simulink model "CIFB2"  (R2022b)
settings: Solver=FixedStepDiscrete  StartTime=0.0  StopTime=0.01  RelTol=1e-3
libraries: dspsrcs4 x1
settings Model: Creator=ASAA  LastModifiedBy=ASAA

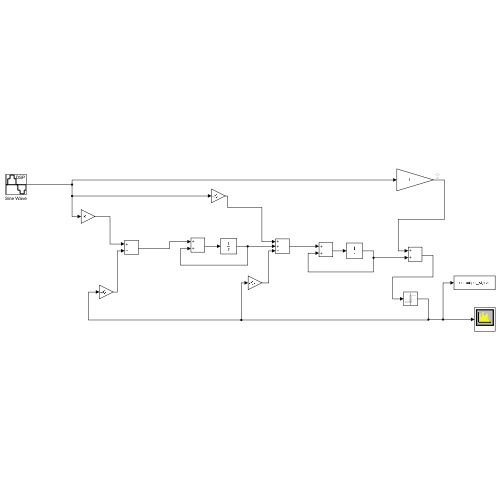
[thumbnail: Simulink's stored preview of the top-level diagram]
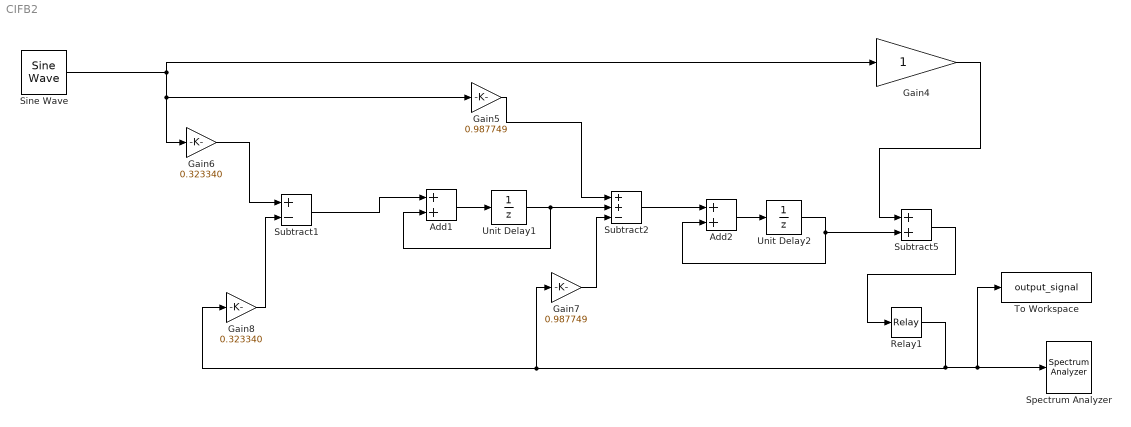
== system CIFB2 ==
  Add1 : Sum
  Add2 : Sum
  Gain4 : Gain
  Gain5 : Gain  Gain=0.987749
  Gain6 : Gain  Gain=0.323340
  Gain7 : Gain  Gain=0.987749
  Gain8 : Gain  Gain=0.323340
  Relay1 : Relay  OffOutputValue=-1
  Sine Wave : dspsrcs4/Sine Wave  Amplitude=0.63  Frequency=100e3  Phase=0  SampleMode=Discrete  OutComplex=Real  CompMethod=Trigonometric fcn  TableSize=Speed  SampleTime=1e-8  SamplesPerFrame=1  ResetState=Restart at time zero  OutputFrames=off  dataType=double  wordLen=16  udDataType=sfix(16)  fracBitsMode=Best precision  numFracBits=15  OutDataTypeStr=double  LastOutDataTypeStr=double
  Spectrum Analyzer : SpectrumAnalyzer
  Subtract1 : Sum  Inputs=+-
  Subtract2 : Sum  Inputs=++-
  Subtract5 : Sum
  To Workspace : ToWorkspace  VariableName=output_signal  SaveFormat=Timeseries  SampleTime=-1
  Unit Delay1 : UnitDelay  SampleTime=1/100e6  HasFrameUpgradeWarning=on
  Unit Delay2 : UnitDelay  SampleTime=1/100e6  HasFrameUpgradeWarning=on
  wires:
  Gain7/1 -> Subtract2/3
  Gain8/1 -> Subtract1/2
  Gain4/1 -> Subtract5/1
  Add2/1 -> Unit Delay2/1
  Add1/1 -> Unit Delay1/1
  Unit Delay1/1 -> Subtract2/2, Add1/2
  Unit Delay2/1 -> Add2/2, Subtract5/2
  Gain6/1 -> Subtract1/1
  Subtract1/1 -> Add1/1
  Gain5/1 -> Subtract2/1
  Subtract5/1 -> Relay1/1
  Subtract2/1 -> Add2/1
  Relay1/1 -> Gain8/1, Gain7/1, To Workspace/1, Spectrum Analyzer/1
  Sine Wave/1 -> Gain5/1, Gain6/1, Gain4/1
